simulink model "hbm"  (R2021a)
settings: Solver=VariableStepAuto  StartTime=0.0  StopTime=10.0  RelTol=1e-3
libraries: xbsIndex_r4 x291
(part 1 of 2)
settings Model: Creator=aisaacson  LastModifiedBy=aisaacson

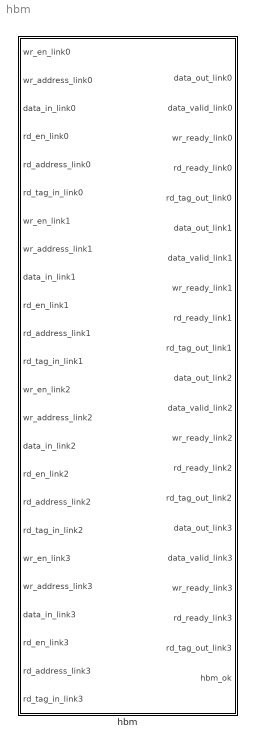
== system hbm ==
  hbm : Subsystem  Tag=xps:hbm  mask(hbm){mem_bank=0, sim_depth=15, sim_latency=5, sim_rand=on}
      mask prompts: mem_bank "Memory Bank"; sim_depth "Depth (2^?)"; sim_latency "Latency"; sim_rand "Randomise"
      mask help: Interface to HBM
      mask init:
      | hbm_mask(gcb);
      | 
      | if sim_rand
      |     %sprintf('sim_rand 1')
      |     set_param([gcb, '/sim_mem1'], 'randread', 'on')   
      |     set_param([gcb, '/sim_mem2'], 'randread', 'on')
      |     set_param([gcb, '/sim_mem3'], 'randread', 'on')
      |     set_param([gcb, '/sim_mem4'], 'randread', 'on')
      |     
      | else
      |     %sprintf('sim_rand 0')
      |     set_param([gcb, '/sim_mem1'], 'randread', 'off')
      |     set_param([gcb, '/sim_mem2'], 'randread', 'off')
      |     set_param([gcb, '/sim_mem3'], 'randread', 'off')
      |     set_param([gcb, '/sim_mem4'], 'randread', 'off')
      | end
      mask TypeOptions mem_bank: 0 | 1
      mask DialogControl Container6 Prompt: Parameters
      mask DialogControl Container7 Prompt: Simulation

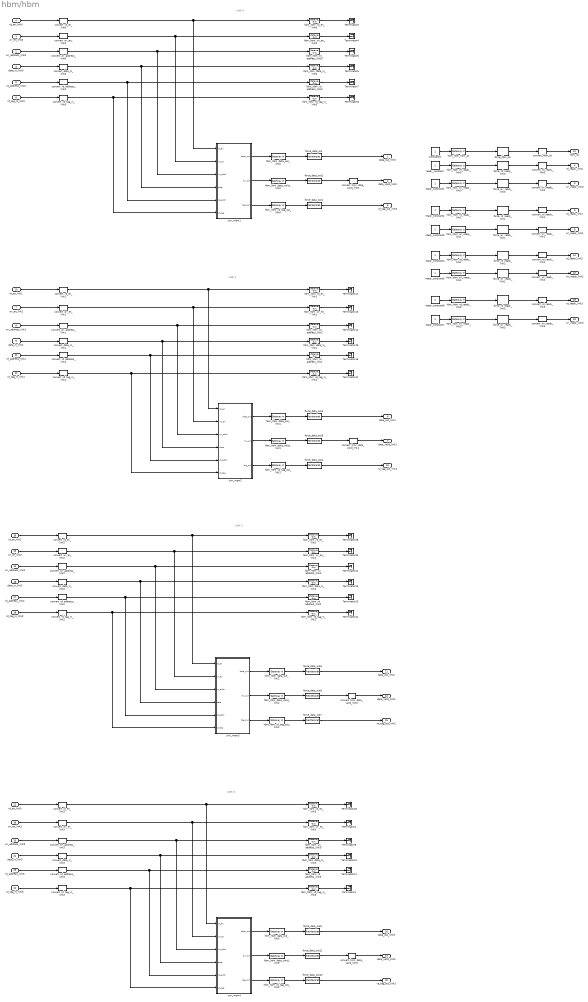
== system hbm/hbm ==
  note: LINK 0
  note: LINK 1
  note: LINK 2
  note: LINK 3
  wr_en_link0 : Inport
  wr_address_link0 : Inport  Port=2
  data_in_link0 : Inport  Port=3
  rd_en_link0 : Inport  Port=4
  rd_address_link0 : Inport  Port=5
  rd_tag_in_link0 : Inport  Port=6
  wr_en_link1 : Inport  Port=7
  wr_address_link1 : Inport  Port=8
  data_in_link1 : Inport  Port=9
  rd_en_link1 : Inport  Port=10
  rd_address_link1 : Inport  Port=11
  rd_tag_in_link1 : Inport  Port=12
  wr_en_link2 : Inport  Port=13
  wr_address_link2 : Inport  Port=14
  data_in_link2 : Inport  Port=15
  rd_en_link2 : Inport  Port=16
  rd_address_link2 : Inport  Port=17
  rd_tag_in_link2 : Inport  Port=18
  wr_en_link3 : Inport  Port=19
  wr_address_link3 : Inport  Port=20
  data_in_link3 : Inport  Port=21
  rd_en_link3 : Inport  Port=22
  rd_address_link3 : Inport  Port=23
  rd_tag_in_link3 : Inport  Port=24
  Constant3 : Constant
  Terminator{1..24} (24 alike) : Terminator
  convert_data_in_link{0..3} (4 alike) : xbsIndex_r4/Convert  gui_display_data_type=Fixed-point  arith_type=Unsigned  n_bits=256  bin_pt=0  float_type=Single  exp_bits=8  fraction_bits=24  quantization=Truncate  overflow=Wrap  en=off  latency=0  pipeline=off  dbl_ovrd=off  block_type=convert
      settings: xl_area=[0, 0, 0, 0, 0, 0, 0]
  convert_hbm_ok : xbsIndex_r4/Convert  gui_display_data_type=Fixed-point  arith_type=Boolean  n_bits=36  bin_pt=0  float_type=Single  exp_bits=8  fraction_bits=24  quantization=Truncate  overflow=Wrap  en=off  latency=0  pipeline=off  dbl_ovrd=off  block_type=convert
      settings: xl_area=[0, 0, 0, 0, 0, 0, 0]
  convert_hmc_data_valid_link{0..3} (4 alike) : xbsIndex_r4/Convert  gui_display_data_type=Boolean  arith_type=Boolean  n_bits=36  bin_pt=0  float_type=Single  exp_bits=8  fraction_bits=24  quantization=Truncate  overflow=Wrap  en=off  latency=0  pipeline=off  dbl_ovrd=off  block_type=convert
      settings: xl_area=[0, 0, 0, 0, 0, 0, 0]
  convert_rd_address_link{0..3} (4 alike) : xbsIndex_r4/Convert  gui_display_data_type=Fixed-point  arith_type=Unsigned  n_bits=27  bin_pt=0  float_type=Single  exp_bits=8  fraction_bits=24  quantization=Truncate  overflow=Wrap  en=off  latency=0  pipeline=off  dbl_ovrd=off  block_type=convert
      settings: xl_area=[0, 0, 0, 0, 0, 0, 0]
  convert_rd_en_link{0..3} (4 alike) : xbsIndex_r4/Convert  gui_display_data_type=Fixed-point  arith_type=Boolean  n_bits=32  bin_pt=0  float_type=Single  exp_bits=8  fraction_bits=24  quantization=Truncate  overflow=Wrap  en=off  latency=0  pipeline=off  dbl_ovrd=off  block_type=convert
      settings: xl_area=[0, 0, 0, 0, 0, 0, 0]
  convert_rd_ready_link{0..3} (4 alike) : xbsIndex_r4/Convert  gui_display_data_type=Fixed-point  arith_type=Boolean  n_bits=36  bin_pt=0  float_type=Single  exp_bits=8  fraction_bits=24  quantization=Truncate  overflow=Wrap  en=off  latency=0  pipeline=off  dbl_ovrd=off  block_type=convert
      settings: xl_area=[0, 0, 0, 0, 0, 0, 0]
  convert_rd_tag_in_link{0..3} (4 alike) : xbsIndex_r4/Convert  gui_display_data_type=Fixed-point  arith_type=Unsigned  n_bits=9  bin_pt=0  float_type=Single  exp_bits=8  fraction_bits=24  quantization=Truncate  overflow=Wrap  en=off  latency=0  pipeline=off  dbl_ovrd=off  block_type=convert
      settings: xl_area=[0, 0, 0, 0, 0, 0, 0]
  convert_wr_address_link{0..3} (4 alike) : xbsIndex_r4/Convert  gui_display_data_type=Fixed-point  arith_type=Unsigned  n_bits=27  bin_pt=0  float_type=Single  exp_bits=8  fraction_bits=24  quantization=Truncate  overflow=Wrap  en=off  latency=0  pipeline=off  dbl_ovrd=off  block_type=convert
      settings: xl_area=[0, 0, 0, 0, 0, 0, 0]
  convert_wr_en_link{0..3} (4 alike) : xbsIndex_r4/Convert  gui_display_data_type=Fixed-point  arith_type=Boolean  n_bits=32  bin_pt=0  float_type=Single  exp_bits=8  fraction_bits=24  quantization=Truncate  overflow=Wrap  en=off  latency=0  pipeline=off  dbl_ovrd=off  block_type=convert
      settings: xl_area=[0, 0, 0, 0, 0, 0, 0]
  convert_wr_ready_link{0..3} (4 alike) : xbsIndex_r4/Convert  gui_display_data_type=Fixed-point  arith_type=Boolean  n_bits=36  bin_pt=0  float_type=Single  exp_bits=8  fraction_bits=24  quantization=Truncate  overflow=Wrap  en=off  latency=0  pipeline=off  dbl_ovrd=off  block_type=convert
      settings: xl_area=[0, 0, 0, 0, 0, 0, 0]
  force_data_out{,1..11} (12 alike) : xbsIndex_r4/Reinterpret  force_arith_type=on  arith_type=Unsigned  force_bin_pt=on  bin_pt=0  block_type=reinterpret
      force_data_out settings: infoedit="Changes signal type without altering the binary representation.   You can changed the signal between signed and unsigned, and relocate the binary point.<P><P>Hardware notes: In hardware this block costs nothing.<P><P>Example:  Suppose the input is 6 bits wide, signed, with 2 fractional bits, and the output is forced to unsigned with 0 fractional bits.  Then an input of -2.0 (1110.00 in binary 2's complement) becomes an output of 56 (111000 in binary)."  block_version=9.1.01
      force_data_out1 settings: block_version=9.1.01
      force_data_out10 settings: block_version=9.1.01
      force_data_out11 settings: block_version=9.1.01
      force_data_out2 settings: block_version=9.1.01
      force_data_out3 settings: infoedit="Changes signal type without altering the binary representation.   You can changed the signal between signed and unsigned, and relocate the binary point.<P><P>Hardware notes: In hardware this block costs nothing.<P><P>Example:  Suppose the input is 6 bits wide, signed, with 2 fractional bits, and the output is forced to unsigned with 0 fractional bits.  Then an input of -2.0 (1110.00 in binary 2's complement) becomes an output of 56 (111000 in binary)."  block_version=9.1.01
      force_data_out4 settings: block_version=9.1.01
      force_data_out5 settings: block_version=9.1.01
      force_data_out6 settings: infoedit="Changes signal type without altering the binary representation.   You can changed the signal between signed and unsigned, and relocate the binary point.<P><P>Hardware notes: In hardware this block costs nothing.<P><P>Example:  Suppose the input is 6 bits wide, signed, with 2 fractional bits, and the output is forced to unsigned with 0 fractional bits.  Then an input of -2.0 (1110.00 in binary 2's complement) becomes an output of 56 (111000 in binary)."  block_version=9.1.01
      force_data_out7 settings: block_version=9.1.01
      force_data_out8 settings: block_version=9.1.01
      force_data_out9 settings: infoedit="Changes signal type without altering the binary representation.   You can changed the signal between signed and unsigned, and relocate the binary point.<P><P>Hardware notes: In hardware this block costs nothing.<P><P>Example:  Suppose the input is 6 bits wide, signed, with 2 fractional bits, and the output is forced to unsigned with 0 fractional bits.  Then an input of -2.0 (1110.00 in binary 2's complement) becomes an output of 56 (111000 in binary)."  block_version=9.1.01
  force_hbm_ok : xbsIndex_r4/Reinterpret  force_arith_type=on  arith_type=Unsigned  force_bin_pt=on  bin_pt=0  block_type=reinterpret
      settings: infoedit="Changes signal type without altering the binary representation.   You can changed the signal between signed and unsigned, and relocate the binary point.<P><P>Hardware notes: In hardware this block costs nothing.<P><P>Example:  Suppose the input is 6 bits wide, signed, with 2 fractional bits, and the output is forced to unsigned with 0 fractional bits.  Then an input of -2.0 (1110.00 in binary 2's complement) becomes an output of 56 (111000 in binary)."  block_version=9.1.01
  force_rd_ready_link{0..3} (4 alike) : xbsIndex_r4/Reinterpret  force_arith_type=on  arith_type=Unsigned  force_bin_pt=on  bin_pt=0  block_type=reinterpret
      settings: infoedit="Changes signal type without altering the binary representation.   You can changed the signal between signed and unsigned, and relocate the binary point.<P><P>Hardware notes: In hardware this block costs nothing.<P><P>Example:  Suppose the input is 6 bits wide, signed, with 2 fractional bits, and the output is forced to unsigned with 0 fractional bits.  Then an input of -2.0 (1110.00 in binary 2's complement) becomes an output of 56 (111000 in binary)."  block_version=9.1.01
  force_wr_ready_link{0..3} (4 alike) : xbsIndex_r4/Reinterpret  force_arith_type=on  arith_type=Unsigned  force_bin_pt=on  bin_pt=0  block_type=reinterpret
      settings: infoedit="Changes signal type without altering the binary representation.   You can changed the signal between signed and unsigned, and relocate the binary point.<P><P>Hardware notes: In hardware this block costs nothing.<P><P>Example:  Suppose the input is 6 bits wide, signed, with 2 fractional bits, and the output is forced to unsigned with 0 fractional bits.  Then an input of -2.0 (1110.00 in binary 2's complement) becomes an output of 56 (111000 in binary)."  block_version=9.1.01
  hbm_hbm_data_in_link{0..3} (4 alike) : xbsIndex_r4/Gateway Out  inherit_from_input=off  hdl_port=on  rows=1  columns=1  UseAsDAC=off  DACChannel='1'  interface=None  automatic_assignment=on  address_offset=hex2dec('00')  intf_name=''  intf_description=''  timing_constraint=None  locs_specified=off  LOCs={}  io_standard={}  block_type=gatewayout
      settings: infoedit="Gateway out block.  Converts Xilinx fixed point inputs into ouputs of type Simulink integer, double, or fixed point.<P><P>Hardware notes:  In hardware these blocks become top level output ports or are discarded, depending on how they are configured."  xl_area=[0, 0, 0, 0, 0, 0, 0]
  hbm_hbm_data_out_link{0..3} (4 alike) : xbsIndex_r4/Gateway In  gui_display_data_type=Fixed-point  arith_type=Unsigned  n_bits=256  bin_pt=0  preci_type=Single  exp_width=8  frac_width=24  rows=1  columns=1  quantization=Truncate  overflow=Wrap  period=1  UseAsADC=off  ADCChannel='1'  interface=None  automatic_assignment=on  address_offset=hex2dec('00')  intf_name=''  intf_description=''  default_value=0  timing_constraint=None  locs_specified=off  LOCs={}  io_standard={}  inherit_from_input=off  hdl_port=on  dbl_ovrd=off  block_type=gatewayin
      settings: xl_area=[0, 0, 0, 0, 0, 0, 0]
  hbm_hbm_data_valid_link{0..3} (4 alike) : xbsIndex_r4/Gateway In  gui_display_data_type=Boolean  arith_type=Boolean  n_bits=9  bin_pt=0  preci_type=Single  exp_width=8  frac_width=24  rows=1  columns=1  quantization=Truncate  overflow=Wrap  period=1  UseAsADC=off  ADCChannel='1'  interface=None  automatic_assignment=on  address_offset=hex2dec('00')  intf_name=''  intf_description=''  default_value=0  timing_constraint=None  locs_specified=off  LOCs={}  io_standard={}  inherit_from_input=off  hdl_port=on  dbl_ovrd=off  block_type=gatewayin
      settings: xl_area=[0, 0, 0, 0, 0, 0, 0]
  hbm_hbm_hbm_ok : xbsIndex_r4/Gateway In  gui_display_data_type=Fixed-point  arith_type=Boolean  n_bits=1  bin_pt=0  preci_type=Single  exp_width=8  frac_width=24  rows=1  columns=1  quantization=Truncate  overflow=Wrap  period=1  UseAsADC=off  ADCChannel='1'  interface=None  automatic_assignment=on  address_offset=hex2dec('00')  intf_name=''  intf_description=''  default_value=0  timing_constraint=None  locs_specified=off  LOCs={}  io_standard={}  inherit_from_input=off  hdl_port=on  dbl_ovrd=off  block_type=gatewayin
      settings: infoedit="Gateway in block.  Converts inputs of type Simulink integer, double and fixed point to  Xilinx fixed point type.<P><P>Hardware notes:  In hardware these blocks become top level input ports."  xl_area=[0, 0, 0, 0, 0, 0, 0]
  hbm_hbm_rd_address_link{0..3} (4 alike) : xbsIndex_r4/Gateway Out  inherit_from_input=off  hdl_port=on  rows=1  columns=1  UseAsDAC=off  DACChannel='1'  interface=None  automatic_assignment=on  address_offset=hex2dec('00')  intf_name=''  intf_description=''  timing_constraint=None  locs_specified=off  LOCs={}  io_standard={}  block_type=gatewayout
      hbm_hbm_rd_address_link0 settings: infoedit="Gateway out block.  Converts Xilinx fixed point inputs into ouputs of type Simulink integer, double, or fixed point.<P><P>Hardware notes:  In hardware these blocks become top level output ports or are discarded, depending on how they are configured."  xl_area=[0, 0, 0, 0, 0, 0, 0]
      hbm_hbm_rd_address_link1 settings: xl_area=[0, 0, 0, 0, 0, 0, 0]
      hbm_hbm_rd_address_link2 settings: infoedit="Gateway out block.  Converts Xilinx fixed point inputs into ouputs of type Simulink integer, double, or fixed point.<P><P>Hardware notes:  In hardware these blocks become top level output ports or are discarded, depending on how they are configured."  xl_area=[0, 0, 0, 0, 0, 0, 0]
      hbm_hbm_rd_address_link3 settings: infoedit="Gateway out block.  Converts Xilinx fixed point inputs into ouputs of type Simulink integer, double, or fixed point.<P><P>Hardware notes:  In hardware these blocks become top level output ports or are discarded, depending on how they are configured."  xl_area=[0, 0, 0, 0, 0, 0, 0]
  hbm_hbm_rd_en_link{0..3} (4 alike) : xbsIndex_r4/Gateway Out  inherit_from_input=off  hdl_port=on  rows=1  columns=1  UseAsDAC=off  DACChannel='1'  interface=None  automatic_assignment=on  address_offset=hex2dec('00')  intf_name=''  intf_description=''  timing_constraint=None  locs_specified=off  LOCs={}  io_standard={}  block_type=gatewayout
      settings: infoedit="Gateway out block.  Converts Xilinx fixed point inputs into ouputs of type Simulink integer, double, or fixed point.<P><P>Hardware notes:  In hardware these blocks become top level output ports or are discarded, depending on how they are configured."  xl_area=[0, 0, 0, 0, 0, 0, 0]
  hbm_hbm_rd_ready_link{0..3} (4 alike) : xbsIndex_r4/Gateway In  gui_display_data_type=Fixed-point  arith_type=Boolean  n_bits=36  bin_pt=0  preci_type=Single  exp_width=8  frac_width=24  rows=1  columns=1  quantization=Truncate  overflow=Wrap  period=1  UseAsADC=off  ADCChannel='1'  interface=None  automatic_assignment=on  address_offset=hex2dec('00')  intf_name=''  intf_description=''  default_value=0  timing_constraint=None  locs_specified=off  LOCs={}  io_standard={}  inherit_from_input=off  hdl_port=on  dbl_ovrd=off  block_type=gatewayin
      settings: infoedit="Gateway in block.  Converts inputs of type Simulink integer, double and fixed point to  Xilinx fixed point type.<P><P>Hardware notes:  In hardware these blocks become top level input ports."  xl_area=[0, 0, 0, 0, 0, 0, 0]
  hbm_hbm_rd_tag_in_link{0..3} (4 alike) : xbsIndex_r4/Gateway Out  inherit_from_input=off  hdl_port=on  rows=1  columns=1  UseAsDAC=off  DACChannel='1'  interface=None  automatic_assignment=on  address_offset=hex2dec('00')  intf_name=''  intf_description=''  timing_constraint=None  locs_specified=off  LOCs={}  io_standard={}  block_type=gatewayout
      settings: infoedit="Gateway out block.  Converts Xilinx fixed point inputs into ouputs of type Simulink integer, double, or fixed point.<P><P>Hardware notes:  In hardware these blocks become top level output ports or are discarded, depending on how they are configured."  xl_area=[0, 0, 0, 0, 0, 0, 0]
  hbm_hbm_rd_tag_out_link{0..3} (4 alike) : xbsIndex_r4/Gateway In  gui_display_data_type=Fixed-point  arith_type=Unsigned  n_bits=9  bin_pt=0  preci_type=Single  exp_width=8  frac_width=24  rows=1  columns=1  quantization=Truncate  overflow=Wrap  period=1  UseAsADC=off  ADCChannel='1'  interface=None  automatic_assignment=on  address_offset=hex2dec('00')  intf_name=''  intf_description=''  default_value=0  timing_constraint=None  locs_specified=off  LOCs={}  io_standard={}  inherit_from_input=off  hdl_port=on  dbl_ovrd=off  block_type=gatewayin
      settings: xl_area=[0, 0, 0, 0, 0, 0, 0]
  hbm_hbm_wr_address_link{0..3} (4 alike) : xbsIndex_r4/Gateway Out  inherit_from_input=off  hdl_port=on  rows=1  columns=1  UseAsDAC=off  DACChannel='1'  interface=None  automatic_assignment=on  address_offset=hex2dec('00')  intf_name=''  intf_description=''  timing_constraint=None  locs_specified=off  LOCs={}  io_standard={}  block_type=gatewayout
      settings: infoedit="Gateway out block.  Converts Xilinx fixed point inputs into ouputs of type Simulink integer, double, or fixed point.<P><P>Hardware notes:  In hardware these blocks become top level output ports or are discarded, depending on how they are configured."  xl_area=[0, 0, 0, 0, 0, 0, 0]
  hbm_hbm_wr_en_link{0..3} (4 alike) : xbsIndex_r4/Gateway Out  inherit_from_input=off  hdl_port=on  rows=1  columns=1  UseAsDAC=off  DACChannel='1'  interface=None  automatic_assignment=on  address_offset=hex2dec('00')  intf_name=''  intf_description=''  timing_constraint=None  locs_specified=off  LOCs={}  io_standard={}  block_type=gatewayout
      settings: infoedit="Gateway out block.  Converts Xilinx fixed point inputs into ouputs of type Simulink integer, double, or fixed point.<P><P>Hardware notes:  In hardware these blocks become top level output ports or are discarded, depending on how they are configured."  xl_area=[0, 0, 0, 0, 0, 0, 0]
  hbm_hbm_wr_ready_link{0..3} (4 alike) : xbsIndex_r4/Gateway In  gui_display_data_type=Fixed-point  arith_type=Boolean  n_bits=36  bin_pt=0  preci_type=Single  exp_width=8  frac_width=24  rows=1  columns=1  quantization=Truncate  overflow=Wrap  period=1  UseAsADC=off  ADCChannel='1'  interface=None  automatic_assignment=on  address_offset=hex2dec('00')  intf_name=''  intf_description=''  default_value=0  timing_constraint=None  locs_specified=off  LOCs={}  io_standard={}  inherit_from_input=off  hdl_port=on  dbl_ovrd=off  block_type=gatewayin
      settings: infoedit="Gateway in block.  Converts inputs of type Simulink integer, double and fixed point to  Xilinx fixed point type.<P><P>Hardware notes:  In hardware these blocks become top level input ports."  xl_area=[0, 0, 0, 0, 0, 0, 0]
  ready_constant{,1..7} (8 alike) : Constant
  sim_mem1 : Subsystem  mask{addr_width=sim_depth, sample_rate=1, csp_latency=sim_latency, randread=on}
      mask prompts: addr_width "Address width"; sample_rate "Sample rate"; csp_latency "Latency"; randread "Randomise read results"
      mask init:
      | if randread
      |     %sprintf('randread 1')
      |     set_param([gcb, '/sfunc'], 'randread', 'on')
      | else
      |     %sprintf('randread 0')
      |     set_param([gcb, '/sfunc'], 'randread', 'off')
      | end
  sim_mem2 : Subsystem  mask{addr_width=sim_depth, sample_rate=1, csp_latency=sim_latency, randread=on}
      mask prompts: addr_width "Address width"; sample_rate "Sample rate"; csp_latency "Latency"; randread "Randomise read results"
      mask init:
      | if randread
      |     set_param([gcb, '/sfunc'], 'randread', 'on')
      | else
      |     set_param([gcb, '/sfunc'], 'randread', 'off')
      | end
  sim_mem3 : Subsystem  mask{addr_width=sim_depth, sample_rate=1, csp_latency=sim_latency, randread=on}
      mask prompts: addr_width "Address width"; sample_rate "Sample rate"; csp_latency "Latency"; randread "Randomise read results"
      mask init:
      | if randread
      |     %sprintf('randread 1')
      |     set_param([gcb, '/sfunc'], 'randread', 'on')
      | else
      |     %sprintf('randread 0')
      |     set_param([gcb, '/sfunc'], 'randread', 'off')
      | end
  sim_mem4 : Subsystem  mask{addr_width=sim_depth, sample_rate=1, csp_latency=sim_latency, randread=on}
      mask prompts: addr_width "Address width"; sample_rate "Sample rate"; csp_latency "Latency"; randread "Randomise read results"
      mask init:
      | if randread
      |     set_param([gcb, '/sfunc'], 'randread', 'on')
      | else
      |     set_param([gcb, '/sfunc'], 'randread', 'off')
      | end
  data_out_link0 : Outport  VectorParamsAs1DForOutWhenUnconnected=off
  data_valid_link0 : Outport  Port=2  VectorParamsAs1DForOutWhenUnconnected=off
  wr_ready_link0 : Outport  Port=3  VectorParamsAs1DForOutWhenUnconnected=off
  rd_ready_link0 : Outport  Port=4  VectorParamsAs1DForOutWhenUnconnected=off
  rd_tag_out_link0 : Outport  Port=5  VectorParamsAs1DForOutWhenUnconnected=off
  data_out_link1 : Outport  Port=6  VectorParamsAs1DForOutWhenUnconnected=off
  data_valid_link1 : Outport  Port=7  VectorParamsAs1DForOutWhenUnconnected=off
  wr_ready_link1 : Outport  Port=8  VectorParamsAs1DForOutWhenUnconnected=off
  rd_ready_link1 : Outport  Port=9  VectorParamsAs1DForOutWhenUnconnected=off
  rd_tag_out_link1 : Outport  Port=10  VectorParamsAs1DForOutWhenUnconnected=off
  data_out_link2 : Outport  Port=11  VectorParamsAs1DForOutWhenUnconnected=off
  data_valid_link2 : Outport  Port=12  VectorParamsAs1DForOutWhenUnconnected=off
  wr_ready_link2 : Outport  Port=13  VectorParamsAs1DForOutWhenUnconnected=off
  rd_ready_link2 : Outport  Port=14  VectorParamsAs1DForOutWhenUnconnected=off
  rd_tag_out_link2 : Outport  Port=15  VectorParamsAs1DForOutWhenUnconnected=off
  data_out_link3 : Outport  Port=16  VectorParamsAs1DForOutWhenUnconnected=off
  data_valid_link3 : Outport  Port=17  VectorParamsAs1DForOutWhenUnconnected=off
  wr_ready_link3 : Outport  Port=18  VectorParamsAs1DForOutWhenUnconnected=off
  rd_ready_link3 : Outport  Port=19  VectorParamsAs1DForOutWhenUnconnected=off
  rd_tag_out_link3 : Outport  Port=20  VectorParamsAs1DForOutWhenUnconnected=off
  hbm_ok : Outport  Port=21  VectorParamsAs1DForOutWhenUnconnected=off
  wires:
  convert_hmc_data_valid_link1/1 -> data_valid_link1/1
  convert_hmc_data_valid_link0/1 -> data_valid_link0/1
  force_data_out/1 -> data_out_link0/1
  sim_mem1/1(data_out) -> hbm_hbm_data_out_link0/1
  sim_mem1/3(tag_out) -> hbm_hbm_rd_tag_out_link0/1
  sim_mem2/3(tag_out) -> hbm_hbm_rd_tag_out_link1/1
  sim_mem2/2(dv_out) -> hbm_hbm_data_valid_link1/1
  sim_mem2/1(data_out) -> hbm_hbm_data_out_link1/1
  sim_mem1/2(dv_out) -> hbm_hbm_data_valid_link0/1
  hbm_hbm_rd_en_link1/1 -> Terminator17/1
  rd_en_link1/1 -> convert_rd_en_link1/1
  convert_rd_en_link1/1 -> sim_mem2/1(rd_en), hbm_hbm_rd_en_link1/1
  hbm_hbm_rd_address_link1/1 -> Terminator16/1
  hbm_hbm_data_in_link1/1 -> Terminator15/1
  hbm_hbm_wr_address_link1/1 -> Terminator14/1
  wr_address_link1/1 -> convert_wr_address_link1/1
  convert_wr_address_link1/1 -> sim_mem2/3(wr_addr), hbm_hbm_wr_address_link1/1
  data_in_link1/1 -> convert_data_in_link1/1
  convert_data_in_link1/1 -> hbm_hbm_data_in_link1/1, sim_mem2/4(data)
  rd_address_link1/1 -> convert_rd_address_link1/1
  convert_rd_address_link1/1 -> sim_mem2/5(rd_addr), hbm_hbm_rd_address_link1/1
  hbm_hbm_wr_en_link1/1 -> Terminator13/1
  wr_en_link1/1 -> convert_wr_en_link1/1
  convert_wr_en_link1/1 -> sim_mem2/2(wr_en), hbm_hbm_wr_en_link1/1
  hbm_hbm_rd_tag_in_link1/1 -> Terminator12/1
  rd_tag_in_link1/1 -> convert_rd_tag_in_link1/1
  convert_rd_tag_in_link1/1 -> sim_mem2/6(rd_tag), hbm_hbm_rd_tag_in_link1/1
  force_data_out5/1 -> convert_hmc_data_valid_link1/1
  force_data_out4/1 -> rd_tag_out_link1/1
  force_data_out3/1 -> data_out_link1/1
  hbm_hbm_data_out_link1/1 -> force_data_out3/1
  hbm_hbm_data_valid_link1/1 -> force_data_out5/1
  hbm_hbm_rd_tag_out_link1/1 -> force_data_out4/1
  convert_wr_ready_link1/1 -> wr_ready_link1/1
  hbm_hbm_wr_ready_link1/1 -> force_wr_ready_link1/1
  ready_constant3/1 -> hbm_hbm_wr_ready_link1/1
  force_wr_ready_link1/1 -> convert_wr_ready_link1/1
  convert_rd_ready_link1/1 -> rd_ready_link1/1
  hbm_hbm_rd_ready_link1/1 -> force_rd_ready_link1/1
  ready_constant2/1 -> hbm_hbm_rd_ready_link1/1
  force_rd_ready_link1/1 -> convert_rd_ready_link1/1
  convert_rd_ready_link0/1 -> rd_ready_link0/1
  convert_hbm_ok/1 -> hbm_ok/1
  hbm_hbm_rd_ready_link0/1 -> force_rd_ready_link0/1
  ready_constant/1 -> hbm_hbm_rd_ready_link0/1
  force_rd_ready_link0/1 -> convert_rd_ready_link0/1
  hbm_hbm_hbm_ok/1 -> force_hbm_ok/1
  Constant3/1 -> hbm_hbm_hbm_ok/1
  force_hbm_ok/1 -> convert_hbm_ok/1
  convert_wr_ready_link0/1 -> wr_ready_link0/1
  hbm_hbm_wr_ready_link0/1 -> force_wr_ready_link0/1
  ready_constant1/1 -> hbm_hbm_wr_ready_link0/1
  force_wr_ready_link0/1 -> convert_wr_ready_link0/1
  hbm_hbm_rd_tag_in_link0/1 -> Terminator8/1
  hbm_hbm_rd_address_link0/1 -> Terminator7/1
  hbm_hbm_data_in_link0/1 -> Terminator6/1
  hbm_hbm_wr_address_link0/1 -> Terminator5/1
  hbm_hbm_wr_en_link0/1 -> Terminator4/1
  hbm_hbm_rd_en_link0/1 -> Terminator3/1
  rd_tag_in_link0/1 -> convert_rd_tag_in_link0/1
  convert_rd_tag_in_link0/1 -> sim_mem1/6(rd_tag), hbm_hbm_rd_tag_in_link0/1
  rd_en_link0/1 -> convert_rd_en_link0/1
  convert_rd_en_link0/1 -> sim_mem1/1(rd_en), hbm_hbm_rd_en_link0/1
  wr_en_link0/1 -> convert_wr_en_link0/1
  convert_wr_en_link0/1 -> sim_mem1/2(wr_en), hbm_hbm_wr_en_link0/1
  wr_address_link0/1 -> convert_wr_address_link0/1
  convert_wr_address_link0/1 -> sim_mem1/3(wr_addr), hbm_hbm_wr_address_link0/1
  data_in_link0/1 -> convert_data_in_link0/1
  convert_data_in_link0/1 -> hbm_hbm_data_in_link0/1, sim_mem1/4(data)
  rd_address_link0/1 -> convert_rd_address_link0/1
  convert_rd_address_link0/1 -> sim_mem1/5(rd_addr), hbm_hbm_rd_address_link0/1
  force_data_out2/1 -> convert_hmc_data_valid_link0/1
  force_data_out1/1 -> rd_tag_out_link0/1
  hbm_hbm_data_out_link0/1 -> force_data_out/1
  hbm_hbm_data_valid_link0/1 -> force_data_out2/1
  hbm_hbm_rd_tag_out_link0/1 -> force_data_out1/1
  force_wr_ready_link2/1 -> convert_wr_ready_link2/1
  ready_constant5/1 -> hbm_hbm_wr_ready_link2/1
  hbm_hbm_wr_ready_link2/1 -> force_wr_ready_link2/1
  convert_wr_ready_link2/1 -> wr_ready_link2/1
  force_rd_ready_link2/1 -> convert_rd_ready_link2/1
  ready_constant4/1 -> hbm_hbm_rd_ready_link2/1
  hbm_hbm_rd_ready_link2/1 -> force_rd_ready_link2/1
  convert_rd_ready_link2/1 -> rd_ready_link2/1
  force_rd_ready_link3/1 -> convert_rd_ready_link3/1
  ready_constant6/1 -> hbm_hbm_rd_ready_link3/1
  hbm_hbm_rd_ready_link3/1 -> force_rd_ready_link3/1
  convert_rd_ready_link3/1 -> rd_ready_link3/1
  force_wr_ready_link3/1 -> convert_wr_ready_link3/1
  ready_constant7/1 -> hbm_hbm_wr_ready_link3/1
  hbm_hbm_wr_ready_link3/1 -> force_wr_ready_link3/1
  convert_wr_ready_link3/1 -> wr_ready_link3/1
  hbm_hbm_rd_tag_out_link2/1 -> force_data_out7/1
  hbm_hbm_data_valid_link2/1 -> force_data_out8/1
  hbm_hbm_data_out_link2/1 -> force_data_out6/1
  force_data_out7/1 -> rd_tag_out_link2/1
  force_data_out8/1 -> convert_hmc_data_valid_link2/1
  convert_rd_address_link2/1 -> hbm_hbm_rd_address_link2/1, sim_mem3/5(rd_addr)
  rd_address_link2/1 -> convert_rd_address_link2/1
  convert_data_in_link2/1 -> hbm_hbm_data_in_link2/1, sim_mem3/4(data)
  data_in_link2/1 -> convert_data_in_link2/1
  convert_wr_address_link2/1 -> hbm_hbm_wr_address_link2/1, sim_mem3/3(wr_addr)
  wr_address_link2/1 -> convert_wr_address_link2/1
  convert_wr_en_link2/1 -> hbm_hbm_wr_en_link2/1, sim_mem3/2(wr_en)
  wr_en_link2/1 -> convert_wr_en_link2/1
  convert_rd_en_link2/1 -> hbm_hbm_rd_en_link2/1, sim_mem3/1(rd_en)
  rd_en_link2/1 -> convert_rd_en_link2/1
  convert_rd_tag_in_link2/1 -> hbm_hbm_rd_tag_in_link2/1, sim_mem3/6(rd_tag)
  rd_tag_in_link2/1 -> convert_rd_tag_in_link2/1
  hbm_hbm_rd_en_link2/1 -> Terminator19/1
  hbm_hbm_wr_en_link2/1 -> Terminator20/1
  hbm_hbm_wr_address_link2/1 -> Terminator21/1
  hbm_hbm_data_in_link2/1 -> Terminator22/1
  hbm_hbm_rd_address_link2/1 -> Terminator23/1
  hbm_hbm_rd_tag_in_link2/1 -> Terminator24/1
  hbm_hbm_rd_tag_out_link3/1 -> force_data_out10/1
  hbm_hbm_data_valid_link3/1 -> force_data_out11/1
  hbm_hbm_data_out_link3/1 -> force_data_out9/1
  force_data_out9/1 -> data_out_link3/1
  force_data_out10/1 -> rd_tag_out_link3/1
  force_data_out11/1 -> convert_hmc_data_valid_link3/1
  convert_rd_tag_in_link3/1 -> hbm_hbm_rd_tag_in_link3/1, sim_mem4/6(rd_tag)
  rd_tag_in_link3/1 -> convert_rd_tag_in_link3/1
  hbm_hbm_rd_tag_in_link3/1 -> Terminator1/1
  convert_wr_en_link3/1 -> hbm_hbm_wr_en_link3/1, sim_mem4/2(wr_en)
  wr_en_link3/1 -> convert_wr_en_link3/1
  hbm_hbm_wr_en_link3/1 -> Terminator2/1
  convert_rd_address_link3/1 -> hbm_hbm_rd_address_link3/1, sim_mem4/5(rd_addr)
  rd_address_link3/1 -> convert_rd_address_link3/1
  convert_data_in_link3/1 -> hbm_hbm_data_in_link3/1, sim_mem4/4(data)
  data_in_link3/1 -> convert_data_in_link3/1
  convert_wr_address_link3/1 -> hbm_hbm_wr_address_link3/1, sim_mem4/3(wr_addr)
  wr_address_link3/1 -> convert_wr_address_link3/1
  hbm_hbm_wr_address_link3/1 -> Terminator9/1
  hbm_hbm_data_in_link3/1 -> Terminator10/1
  hbm_hbm_rd_address_link3/1 -> Terminator11/1
  convert_rd_en_link3/1 -> hbm_hbm_rd_en_link3/1, sim_mem4/1(rd_en)
  rd_en_link3/1 -> convert_rd_en_link3/1
  hbm_hbm_rd_en_link3/1 -> Terminator18/1
  sim_mem3/2(dv_out) -> hbm_hbm_data_valid_link2/1
  sim_mem4/1(data_out) -> hbm_hbm_data_out_link3/1
  sim_mem4/2(dv_out) -> hbm_hbm_data_valid_link3/1
  sim_mem4/3(tag_out) -> hbm_hbm_rd_tag_out_link3/1
  sim_mem3/3(tag_out) -> hbm_hbm_rd_tag_out_link2/1
  sim_mem3/1(data_out) -> hbm_hbm_data_out_link2/1
  force_data_out6/1 -> data_out_link2/1
  convert_hmc_data_valid_link2/1 -> data_valid_link2/1
  convert_hmc_data_valid_link3/1 -> data_valid_link3/1

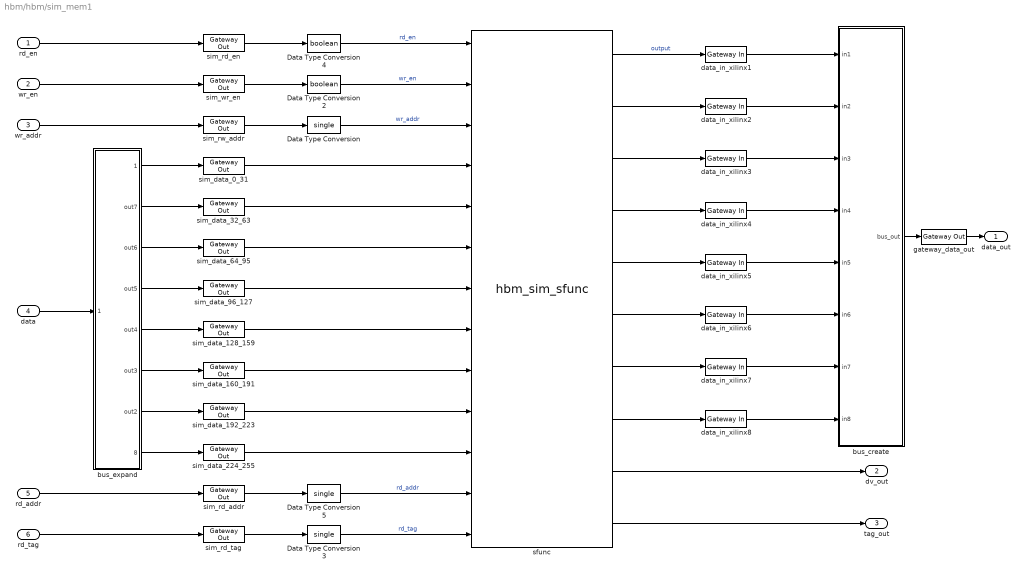
== system hbm/hbm/sim_mem1 ==
  rd_en : Inport
  wr_en : Inport  Port=2
  wr_addr : Inport  Port=3
  data : Inport  Port=4
  rd_addr : Inport  Port=5
  rd_tag : Inport  Port=6
  Data Type Conversion : DataTypeConversion  OutDataTypeStr=single
  Data Type Conversion2 : DataTypeConversion  OutDataTypeStr=boolean
  Data Type Conversion3 : DataTypeConversion  OutDataTypeStr=single
  Data Type Conversion4 : DataTypeConversion  OutDataTypeStr=boolean
  Data Type Conversion5 : DataTypeConversion  OutDataTypeStr=single
  bus_create : Subsystem  AncestorBlock=casper_library_flow_control/bus_create  mask(bus_create){inputNum=8}
      mask prompts: inputNum "Number of inputs:"
      mask init:
      | bus_create_init(gcb,...
      |     'inputNum', inputNum);
  bus_expand : Subsystem  AncestorBlock=casper_library_flow_control/bus_expand  mask(bus_expand){mode=divisions of equal size, outputNum=8, outputWidth=32, outputBinaryPt=0, outputArithmeticType=0, show_format=off, outputToWorkspace=off, variablePrefix=out, outputToModelAsWell=on}
      mask prompts: outputNum "Number of outputs:"; outputWidth "Output width:"; outputBinaryPt "Output binary point position:"; outputArithmeticType "Output arithmetic type (ufix=0, fix=1, bool=2):"; show_format "Print format string?"; outputToWorkspace "Output to workspace?"; variablePrefix "Variable name prefix:"; outputToModelAsWell "Output to model as well?"
      mask help:
      | Expands a 'bus' made using a bus_create or Xilinx
      | concat block.
      | The input will be divided into the specified number
      | of outputs with the specified arithmetic types.
      | Divisions are made from most significant bit.
      mask init:
      | bus_expand_init(gcb,...
      |     'mode', mode, ...
      |     'outputNum', outputNum, ...
      |     'outputWidth', outputWidth, ...
      |     'outputBinaryPt', outputBinaryPt, ...
      |     'outputArithmeticType', outputArithmeticType, ...
      |     'show_format', show_format, ...
      |     'outputToWorkspace', outputToWorkspace, ...
      |     'variablePrefix', variablePrefix, ...
      |     'outputToModelAsWell', outputToModelAsWell);
      settings: AttributesFormatString=8 outputs
      mask TypeOptions mode: divisions of equal size | divisions of arbitrary size
      mask Callback mode: bus_expand_callback();
      mask Callback outputWidth: bus_expand_callback();
      mask Callback outputToWorkspace: bus_expand_callback();
  data_in_xilinx{1..8} (8 alike) : xbsIndex_r4/Gateway In  gui_display_data_type=Fixed-point  arith_type=Unsigned  n_bits=32  bin_pt=0  preci_type=Single  exp_width=8  frac_width=24  rows=1  columns=1  quantization=Truncate  overflow=Wrap  period=1  UseAsADC=off  ADCChannel='1'  interface=None  automatic_assignment=on  address_offset=hex2dec('00')  intf_name=''  intf_description=''  default_value=0  timing_constraint=None  locs_specified=off  LOCs={}  io_standard={}  inherit_from_input=off  hdl_port=on  dbl_ovrd=off  block_type=gatewayin
      settings: xl_area=[0, 0, 0, 0, 0, 0, 0]
  gateway_data_out : xbsIndex_r4/Gateway Out  inherit_from_input=off  hdl_port=off  rows=1  columns=1  UseAsDAC=off  DACChannel='1'  interface=None  automatic_assignment=on  address_offset=hex2dec('00')  intf_name=''  intf_description=''  timing_constraint=None  locs_specified=off  LOCs={}  io_standard={}  block_type=gatewayout
  sfunc : M-S-Function  FunctionName=hbm_sim_sfunc  Parameters=depth_bits, latency, randread  mask{depth_bits=addr_width, latency=csp_latency, randread=on}
      mask prompts: depth_bits "Depth (2^?):"; latency "Latency (>=1):"; randread "Randomise read results"
      mask init:
      | % if randread
      | %     sprintf('sfunc randread 1')
      | % else
      | %     sprintf('sfunc randread 0')
      | % end
      mask Callback latency:
      | latency = str2double(get_param(gcb, 'latency'));
      | if latency < 1
      |     errordlg('Cannot have latency less than one.');
      |     set_param(gcb, 'latency', '1');
      | end
  sim_data_0_31 : xbsIndex_r4/Gateway Out  inherit_from_input=off  hdl_port=off  rows=1  columns=1  UseAsDAC=off  DACChannel='1'  interface=None  automatic_assignment=on  address_offset=hex2dec('00')  intf_name=''  intf_description=''  timing_constraint=None  locs_specified=off  LOCs={}  io_standard={}  block_type=gatewayout
  sim_data_128_159 : xbsIndex_r4/Gateway Out  inherit_from_input=off  hdl_port=off  rows=1  columns=1  UseAsDAC=off  DACChannel='1'  interface=None  automatic_assignment=on  address_offset=hex2dec('00')  intf_name=''  intf_description=''  timing_constraint=None  locs_specified=off  LOCs={}  io_standard={}  block_type=gatewayout
  sim_data_160_191 : xbsIndex_r4/Gateway Out  inherit_from_input=off  hdl_port=off  rows=1  columns=1  UseAsDAC=off  DACChannel='1'  interface=None  automatic_assignment=on  address_offset=hex2dec('00')  intf_name=''  intf_description=''  timing_constraint=None  locs_specified=off  LOCs={}  io_standard={}  block_type=gatewayout
  sim_data_192_223 : xbsIndex_r4/Gateway Out  inherit_from_input=off  hdl_port=off  rows=1  columns=1  UseAsDAC=off  DACChannel='1'  interface=None  automatic_assignment=on  address_offset=hex2dec('00')  intf_name=''  intf_description=''  timing_constraint=None  locs_specified=off  LOCs={}  io_standard={}  block_type=gatewayout
  sim_data_224_255 : xbsIndex_r4/Gateway Out  inherit_from_input=off  hdl_port=off  rows=1  columns=1  UseAsDAC=off  DACChannel='1'  interface=None  automatic_assignment=on  address_offset=hex2dec('00')  intf_name=''  intf_description=''  timing_constraint=None  locs_specified=off  LOCs={}  io_standard={}  block_type=gatewayout
  sim_data_32_63 : xbsIndex_r4/Gateway Out  inherit_from_input=off  hdl_port=off  rows=1  columns=1  UseAsDAC=off  DACChannel='1'  interface=None  automatic_assignment=on  address_offset=hex2dec('00')  intf_name=''  intf_description=''  timing_constraint=None  locs_specified=off  LOCs={}  io_standard={}  block_type=gatewayout
  sim_data_64_95 : xbsIndex_r4/Gateway Out  inherit_from_input=off  hdl_port=off  rows=1  columns=1  UseAsDAC=off  DACChannel='1'  interface=None  automatic_assignment=on  address_offset=hex2dec('00')  intf_name=''  intf_description=''  timing_constraint=None  locs_specified=off  LOCs={}  io_standard={}  block_type=gatewayout
  sim_data_96_127 : xbsIndex_r4/Gateway Out  inherit_from_input=off  hdl_port=off  rows=1  columns=1  UseAsDAC=off  DACChannel='1'  interface=None  automatic_assignment=on  address_offset=hex2dec('00')  intf_name=''  intf_description=''  timing_constraint=None  locs_specified=off  LOCs={}  io_standard={}  block_type=gatewayout
  sim_rd_addr : xbsIndex_r4/Gateway Out  inherit_from_input=off  hdl_port=off  rows=1  columns=1  UseAsDAC=off  DACChannel='1'  interface=None  automatic_assignment=on  address_offset=hex2dec('00')  intf_name=''  intf_description=''  timing_constraint=None  locs_specified=off  LOCs={}  io_standard={}  block_type=gatewayout
  sim_rd_en : xbsIndex_r4/Gateway Out  inherit_from_input=off  hdl_port=off  rows=1  columns=1  UseAsDAC=off  DACChannel='1'  interface=None  automatic_assignment=on  address_offset=hex2dec('00')  intf_name=''  intf_description=''  timing_constraint=None  locs_specified=off  LOCs={}  io_standard={}  block_type=gatewayout
  sim_rd_tag : xbsIndex_r4/Gateway Out  inherit_from_input=off  hdl_port=off  rows=1  columns=1  UseAsDAC=off  DACChannel='1'  interface=None  automatic_assignment=on  address_offset=hex2dec('00')  intf_name=''  intf_description=''  timing_constraint=None  locs_specified=off  LOCs={}  io_standard={}  block_type=gatewayout
  sim_rw_addr : xbsIndex_r4/Gateway Out  inherit_from_input=off  hdl_port=off  rows=1  columns=1  UseAsDAC=off  DACChannel='1'  interface=None  automatic_assignment=on  address_offset=hex2dec('00')  intf_name=''  intf_description=''  timing_constraint=None  locs_specified=off  LOCs={}  io_standard={}  block_type=gatewayout
  sim_wr_en : xbsIndex_r4/Gateway Out  inherit_from_input=off  hdl_port=off  rows=1  columns=1  UseAsDAC=off  DACChannel='1'  interface=None  automatic_assignment=on  address_offset=hex2dec('00')  intf_name=''  intf_description=''  timing_constraint=None  locs_specified=off  LOCs={}  io_standard={}  block_type=gatewayout
  data_out : Outport  VectorParamsAs1DForOutWhenUnconnected=off
  dv_out : Outport  Port=2  VectorParamsAs1DForOutWhenUnconnected=off
  tag_out : Outport  Port=3  VectorParamsAs1DForOutWhenUnconnected=off
  wires:
  sfunc/10 -> tag_out/1
  sfunc/9 -> dv_out/1
  gateway_data_out/1 -> data_out/1
  bus_create/1(bus_out) -> gateway_data_out/1
  sim_data_0_31/1 -> sfunc/4
  sim_data_32_63/1 -> sfunc/5
  sim_data_64_95/1 -> sfunc/6
  sim_data_96_127/1 -> sfunc/7
  sim_data_128_159/1 -> sfunc/8
  sim_data_160_191/1 -> sfunc/9
  sim_data_192_223/1 -> sfunc/10
  sim_data_224_255/1 -> sfunc/11
  data/1 -> bus_expand/1(bus_in)
  Data Type Conversion3/1 -> sfunc/13  "rd_tag"
  Data Type Conversion5/1 -> sfunc/12  "rd_addr"
  Data Type Conversion2/1 -> sfunc/2  "wr_en"
  Data Type Conversion/1 -> sfunc/3  "wr_addr"
  sim_wr_en/1 -> Data Type Conversion2/1
  sim_rw_addr/1 -> Data Type Conversion/1
  wr_en/1 -> sim_wr_en/1
  wr_addr/1 -> sim_rw_addr/1
  Data Type Conversion4/1 -> sfunc/1  "rd_en"
  sim_rd_en/1 -> Data Type Conversion4/1
  rd_en/1 -> sim_rd_en/1
  sim_rd_addr/1 -> Data Type Conversion5/1
  rd_addr/1 -> sim_rd_addr/1
  sim_rd_tag/1 -> Data Type Conversion3/1
  rd_tag/1 -> sim_rd_tag/1
  bus_expand/1(msb_out8) -> sim_data_0_31/1
  bus_expand/2(out7) -> sim_data_32_63/1
  bus_expand/3(out6) -> sim_data_64_95/1
  bus_expand/4(out5) -> sim_data_96_127/1
  bus_expand/5(out4) -> sim_data_128_159/1
  bus_expand/6(out3) -> sim_data_160_191/1
  bus_expand/7(out2) -> sim_data_192_223/1
  bus_expand/8(lsb_out1) -> sim_data_224_255/1
  sfunc/1 -> data_in_xilinx1/1  "output"
  data_in_xilinx1/1 -> bus_create/1(in1)
  sfunc/2 -> data_in_xilinx2/1
  data_in_xilinx2/1 -> bus_create/2(in2)
  sfunc/3 -> data_in_xilinx3/1
  data_in_xilinx3/1 -> bus_create/3(in3)
  sfunc/4 -> data_in_xilinx4/1
  data_in_xilinx4/1 -> bus_create/4(in4)
  sfunc/5 -> data_in_xilinx5/1
  data_in_xilinx5/1 -> bus_create/5(in5)
  sfunc/6 -> data_in_xilinx6/1
  data_in_xilinx6/1 -> bus_create/6(in6)
  sfunc/7 -> data_in_xilinx7/1
  data_in_xilinx7/1 -> bus_create/7(in7)
  sfunc/8 -> data_in_xilinx8/1
  data_in_xilinx8/1 -> bus_create/8(in8)
